simulink model "dc_motor_part_1"  (R2026b)
settings: Solver=VariableStepAuto
model workspace (MAT data in the model file):
  Var = 0
  b = 0.0005
  j = 5e-05
  k = 0.2
  l = 0.41
  r = 4
  v = 7.4
settings Model: Creator=Amaan  LastModifiedBy=Amaan

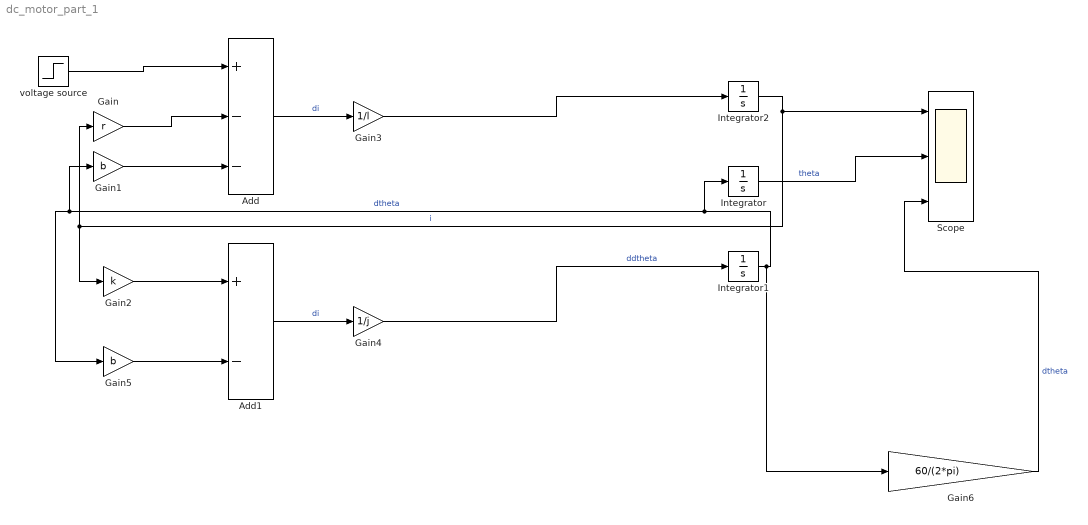
== system dc_motor_part_1 ==
  Add : Sum  Inputs=+--
  Add1 : Sum  Inputs=+-
  Gain : Gain  Gain=r
  Gain1 : Gain  Gain=b
  Gain2 : Gain  Gain=k
  Gain3 : Gain  Gain=1/l
  Gain4 : Gain  Gain=1/j
  Gain5 : Gain  Gain=b
  Gain6 : Gain  Gain=60/(2*pi)
  Integrator : Integrator
  Integrator1 : Integrator
  Integrator2 : Integrator
  Scope : Scope  NumInputPorts=3
      settings: ActiveDisplayYMinimum=-0.93769870745677719  ActiveDisplayYMaximum=8.4392883671109971
  voltage source : Step  FinalValue=v  SampleTime=0
  wires:
  Integrator2/1 -> Gain/1, Gain2/1, Scope/1  "i"
  Integrator1/1 -> Gain6/1, Gain1/1, Gain5/1, Integrator/1  "dtheta"
  Gain4/1 -> Integrator1/1  "ddtheta"
  voltage source/1 -> Add/1
  Gain/1 -> Add/2
  Gain1/1 -> Add/3
  Gain2/1 -> Add1/1
  Add/1 -> Gain3/1  "di"
  Gain3/1 -> Integrator2/1
  Add1/1 -> Gain4/1  "di"
  Gain5/1 -> Add1/2
  Gain6/1 -> Scope/3  "dtheta"
  Integrator/1 -> Scope/2  "theta"
